simulink model "grid_afe_n"  (R2026a)
settings: Solver=ode23tb  StopTime=simlength  FixedStep=tc  MaxStep=glb_time.tc
values from neighbouring files (symbols this model uses):
  afe_ctrl = ctrl_afe_setup(glb_time.ts_afe, grid_emu.omega_grid_nom)    [init_model.m]
  afe_pwm_phase_shift_mod1 = 0    [init_model.m]
  afe_pwm_phase_shift_mod2 = 0    [init_model.m]
  afe_pwm_phase_shift_mod3 = 0    [init_model.m]
  afe_pwm_phase_shift_mod4 = 0    [init_model.m]
  filters = setup_global_filters(glb_time.ts_afe, glb_time.ts_inv, glb_time.ts_dab, glb_time.tc)    [init_model.m]
  frt_data = frt_settings(test_index, test_subindex, asymmetric_error_type,      enable_frt_1, enable_frt_2, start_time_LVRT, deepPOSxi, deepPOSeta, deepNEGxi, deepNEGeta)    [init_model.m]
  glb_time = timing_setup(fpwm_afe, trgo_afe, fpwm_inv, trgo_inv, fpwm_single_phase_inv, trgo_single_phase_inv, fpwm_dab, trgo_dab,      fpwm_psfbc, trgo_psfbc, fpwm_isop_rail, trgo_isop_rail, fpwm_cllc, trgo_cllc, t_measure, tc_factor, tc_decimation, delay_pwm, dead_time_afe,      dead_time_inv, dead_time_single_phase_inv, dead_time_dab, dead_time_psfbc, dead_time_isop_rail, dead_time_cllc)    [init_model.m]
  grid_emu = grid_three_phase_emulator('Dyn11', delta_star, grid_nominal_power, application_voltage, us1, us2, fgrid,                  eq_grid_inductance, eq_grid_resistance, eta, ucc, i1m, p_iron, n1, n2, core_area, core_length, mur,                  up_xi_pu_ref, up_eta_pu_ref, un_xi_pu_ref, un_eta_pu_ref)    [init_model.m]
  i_react_pos_ref_2 = -ixi_ref_mod1*tan(acos(0.95))    [init_model.m]
  i_react_pos_ref_3 = ixi_ref_mod1*tan(acos(0.95))    [init_model.m]
  ixi_ref_mod1 = -0.85    [init_model.m]
  ixi_ref_mod2 = -0.85    [init_model.m]
  ixi_ref_mod3 = -0.85    [init_model.m]
  ixi_ref_mod4 = -0.85    [init_model.m]
  ki_align = 18    [init_model.m]
  kp_align = 0.25    [init_model.m]
  lim_down_align = -0.05    [init_model.m]
  lim_up_align = 0.05    [init_model.m]
  mavarage_filter_frequency_base_order = 2    [init_model.m]
  time_gain_afe_module_1 = 1.0002    [init_model.m]
  time_gain_afe_module_2 = 1.0015    [init_model.m]
  time_gain_afe_module_3 = 0.9988    [init_model.m]
  time_gain_afe_module_4 = 1.0020    (= 1.002)    [init_model.m]
  time_i_react_pos_ref_1 = start_time_LVRT + error_length + 0.335    [init_model.m]
  time_i_react_pos_ref_2 = time_i_react_pos_ref_1 + 0.5    (= 0.5)    [init_model.m]
  u_cm_comp_mod1 = 0    [init_model.m]
  u_cm_comp_mod2 = -1    [init_model.m]
  u_cm_comp_mod3 = -1    [init_model.m]
  u_cm_comp_mod4 = -1    [init_model.m]
undefined symbols (not defined in the file or in its folder): hwdata, magnitude
libraries: fl_lib x113, nesl_utility x75, moving_average_filter x40, moving_average_filter_cc x32, sl_discontinuities x12, linear_double_integrator_observer_ccaller x8, discrete_time_low_pass_filter x4, threephase_inductor_lib x4, dclink_for_two_levels x4, three_phase_pwm_modulator x4, three_phase_inverter_ideal_switch_based_model x4, three_phase_inverter_igbt_advanced_thermal_model x4
(part 6 of 19)

== system grid_afe_n/afe_abc_mod3/AFE_control/afe_control/ig afe quantizzation and one step delay ==
  ig_abc_pu : Inport
  Demux1 : Demux  Outputs=3
  Mux1 : Mux  Inputs=3
  ig afe quantizzation and one step delay : Subsystem
  igd_abc_pu : Outport
  wires:
  Demux1/1 -> ig afe quantizzation and one step delay/1(ig_u_pu)
  Demux1/2 -> ig afe quantizzation and one step delay/2(ig_v_pu)
  ig_abc_pu/1 -> Demux1/1
  Mux1/1 -> igd_abc_pu/1
  Demux1/3 -> ig afe quantizzation and one step delay/3(ig_w_pu)
  ig afe quantizzation and one step delay/2(igd_v_pu) -> Mux1/2
  ig afe quantizzation and one step delay/1(igd_u_pu) -> Mux1/1
  ig afe quantizzation and one step delay/3(igd_w_pu) -> Mux1/3

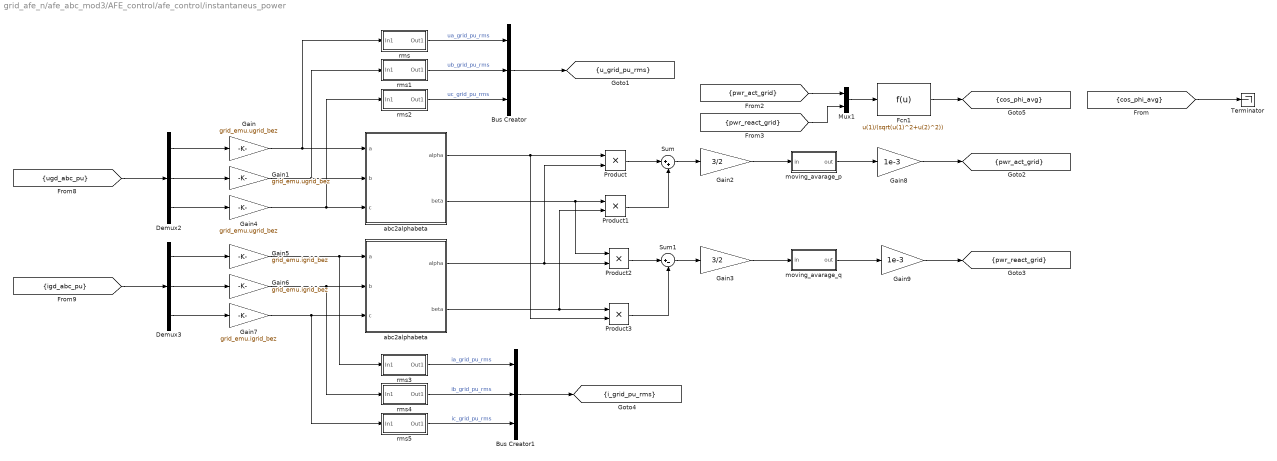
== system grid_afe_n/afe_abc_mod3/AFE_control/afe_control/instantaneus_power ==
  Bus Creator : BusCreator  Inputs=3
  Bus Creator1 : BusCreator  Inputs=3
  Demux2 : Demux  Outputs=3
  Demux3 : Demux  Outputs=3
  Fcn1 : Fcn  Expr=u(1)/(sqrt(u(1)^2+u(2)^2))
  Gain : Gain  Gain=grid_emu.ugrid_bez
  Gain1 : Gain  Gain=grid_emu.ugrid_bez
  Gain2 : Gain  Gain=3/2
  Gain3 : Gain  Gain=3/2
  Gain4 : Gain  Gain=grid_emu.ugrid_bez
  Gain5 : Gain  Gain=grid_emu.igrid_bez
  Gain6 : Gain  Gain=grid_emu.igrid_bez
  Gain7 : Gain  Gain=grid_emu.igrid_bez
  Gain8 : Gain  Gain=1e-3
  Gain9 : Gain  Gain=1e-3
  Mux1 : Mux  Inputs=2
  Product{,1..3} (4 alike) : Product  RndMeth=Zero
  Sum : Sum  Inputs=|++
  Sum1 : Sum  Inputs=|+-
  Terminator : Terminator
  abc2alphabeta : Subsystem
  "abc2alphabeta " : Subsystem
  moving_avarage_p : Subsystem
  moving_avarage_q : Subsystem
  rms : Subsystem
  rms1 : Subsystem
  rms2 : Subsystem
  rms3 : Subsystem
  rms4 : Subsystem
  rms5 : Subsystem
  tag scope: cos_phi_avg=scoped, i_grid_pu_rms=scoped, pwr_act_grid=scoped, pwr_react_grid=scoped, u_grid_pu_rms=scoped
  wires:
  abc2alphabeta/2("beta ") -> Product1/1, Product2/1
  "abc2alphabeta "/2("beta ") -> Product1/2, Product3/1
  abc2alphabeta/1("alpha ") -> Product3/2, Product/1
  "abc2alphabeta "/1("alpha ") -> Product2/2, Product/2
  Product/1 -> Sum/1
  Product1/1 -> Sum/2
  Product2/1 -> Sum1/1
  Product3/1 -> Sum1/2
  Sum1/1 -> Gain3/1
  Sum/1 -> Gain2/1
  Gain2/1 -> moving_avarage_p/1(in)
  Gain3/1 -> moving_avarage_q/1(in)
  [pwr_react_grid] -> Mux1/2
  Mux1/1 -> Fcn1/1
  Fcn1/1 -> [cos_phi_avg]
  [pwr_act_grid] -> Mux1/1
  rms/1(Out1) -> Bus Creator/1  "ua_grid_pu_rms"
  rms2/1(Out1) -> Bus Creator/3  "uc_grid_pu_rms"
  rms1/1(Out1) -> Bus Creator/2  "ub_grid_pu_rms"
  moving_avarage_p/1(out) -> Gain8/1
  moving_avarage_q/1(out) -> Gain9/1
  Demux2/1 -> Gain/1
  Demux2/2 -> Gain1/1
  Demux2/3 -> Gain4/1
  Demux3/1 -> Gain5/1
  Demux3/2 -> Gain6/1
  Demux3/3 -> Gain7/1
  Gain/1 -> rms/1(In1), abc2alphabeta/1(a)
  Gain1/1 -> rms1/1(In1), abc2alphabeta/2(b)
  Gain4/1 -> rms2/1(In1), abc2alphabeta/3(c)
  Gain5/1 -> rms3/1(In1), "abc2alphabeta "/1(a)
  Gain6/1 -> rms4/1(In1), "abc2alphabeta "/2(b)
  Gain7/1 -> rms5/1(In1), "abc2alphabeta "/3(c)
  Gain8/1 -> [pwr_act_grid]
  Gain9/1 -> [pwr_react_grid]
  [ugd_abc_pu] -> Demux2/1
  [igd_abc_pu] -> Demux3/1
  Bus Creator/1 -> [u_grid_pu_rms]
  rms4/1(Out1) -> Bus Creator1/2  "ib_grid_pu_rms"
  rms3/1(Out1) -> Bus Creator1/1  "ia_grid_pu_rms"
  rms5/1(Out1) -> Bus Creator1/3  "ic_grid_pu_rms"
  Bus Creator1/1 -> [i_grid_pu_rms]
  [cos_phi_avg] -> Terminator/1

== system grid_afe_n/afe_abc_mod3/AFE_control/afe_control/interesting scopes ==
  current_sequences_mod1 : Scope  NumInputPorts=4
      settings: ActiveDisplayYMinimum=-1.4062410671621262  ActiveDisplayYMaximum=0.648263540608363  DataLoggingVariableName=ScopeData2
  i_grid_seq_ref : Scope
      settings: ActiveDisplayYMinimum=-1.125  ActiveDisplayYMaximum=0.125
  voltage_sequences_mod1 : Scope  NumInputPorts=4
      settings: ActiveDisplayYMinimum=-1.2405151816982258  ActiveDisplayYMaximum=1.2605257614333911
  wires:
  [v_grid_neg_eta_avg] -> voltage_sequences_mod1/4  "u_grid_neg_eta"
  [i_grid_neg_xi_avg] -> current_sequences_mod1/3  "i_grid_neg_xi"
  [v_grid_pos_eta_avg] -> voltage_sequences_mod1/2  "u_grid_pos_eta"
  [v_grid_neg_xi_avg] -> voltage_sequences_mod1/3  "u_grid_neg_xi"
  [i_grid_pos_xi_avg] -> current_sequences_mod1/1  "i_grid_pos_xi"
  [i_grid_neg_eta_avg] -> current_sequences_mod1/4  "i_grid_neg_eta"
  [v_grid_pos_xi_avg] -> voltage_sequences_mod1/1  "u_grid_pos_xi"
  [i_grid_pos_eta_avg] -> current_sequences_mod1/2  "i_grid_pos_eta"
  [i_grid_seq_ref] -> i_grid_seq_ref/1  "i_grid_seq_ref"

== system grid_afe_n/afe_abc_mod3/AFE_control/afe_control/is afe quantizzation and one step delay ==
  is_abc_pu : Inport
  Demux : Demux  Outputs=3
  Mux : Mux  Inputs=3
  is afe quantizzation and one step delay : Subsystem
  isd_abc_pu : Outport
  wires:
  is afe quantizzation and one step delay/2(isd_v_pu) -> Mux/2
  is_abc_pu/1 -> Demux/1
  is afe quantizzation and one step delay/3(isd_w_pu) -> Mux/3
  is afe quantizzation and one step delay/1(isd_u_pu) -> Mux/1
  Demux/1 -> is afe quantizzation and one step delay/1(is_u_pu)
  Mux/1 -> isd_abc_pu/1
  Demux/3 -> is afe quantizzation and one step delay/3(is_w_pu)
  Demux/2 -> is afe quantizzation and one step delay/2(is_v_pu)

== system grid_afe_n/afe_abc_mod3/AFE_control/afe_control/islanding_mode_detector ==
  gamma : Inport
  alpha : Inport  Port=2
  beta : Inport  Port=3
  Gain : Gain  Gain=7
  MATLAB Function : MATLAB Function  TreatAsAtomicUnit=on
  Terminator : Terminator
  Terminator1 : Terminator
  bounder : MATLAB Function  TreatAsAtomicUnit=on
  moving_avarage_1 : Subsystem
  moving_avarage_2 : Subsystem
  seventh_ugrid_component : Scope  NumInputPorts=2
      settings: ActiveDisplayYMinimum=-0.0034745064787606167  ActiveDisplayYMaximum=0.0074022094547510631  DataLoggingVariableName=ScopeData10
  tag scope: u_7th_eta_avg=scoped, u_7th_xi_avg=scoped
  wires:
  gamma/1 -> Gain/1  "gamma_grid"
  MATLAB Function/1(xi) -> moving_avarage_1/1(u)
  bounder/1(y) -> MATLAB Function/3(gamma)
  Gain/1 -> bounder/1(u)
  alpha/1 -> MATLAB Function/1(alpha)  "u_grid_alpha"
  beta/1 -> MATLAB Function/2(beta)  "u_grid_beta"
  MATLAB Function/2(eta) -> moving_avarage_2/1(u)
  moving_avarage_1/1(y) -> [u_7th_xi_avg], seventh_ugrid_component/1  "u_7th_xi"
  moving_avarage_2/1(y) -> seventh_ugrid_component/2, [u_7th_eta_avg]  "u_7th_eta"
  [u_7th_xi_avg] -> Terminator/1
  [u_7th_eta_avg] -> Terminator1/1

== system grid_afe_n/afe_abc_mod3/AFE_control/afe_control/phase_compensation_1 ==
  local_time : Inport
  master_time : Inport  Port=2
  Zero-Order Hold : ZeroOrderHold  SampleTime=-1
  Zero-Order Hold1 : ZeroOrderHold  SampleTime=-1
  alignment_eval_afe1 : Subsystem
  y : Outport
  wires:
  local_time/1 -> Zero-Order Hold/1
  master_time/1 -> Zero-Order Hold1/1
  alignment_eval_afe1/1(dp) -> y/1
  Zero-Order Hold/1 -> alignment_eval_afe1/1(local_time)
  Zero-Order Hold1/1 -> alignment_eval_afe1/2(master_time)

== system grid_afe_n/afe_abc_mod3/AFE_control/afe_control/space_vector ==
  uab_out : Inport
  Bus Creator : BusCreator  Inputs=3
  Bus Selector : BusSelector  OutputSignals=da,db,dc
  Bus Selector1 : BusSelector  OutputSignals=ualpha_afe,ubeta_afe,ugamma_afe
  C Caller : CCaller  FunctionName=sv_pwm_cm_process_simulink  PortSpecificationStruct="%)30     .    B H   8    (     @         %    \"     8    !     0         %  0 \"0    $    _    07)G3F%M90  4&]R=$YA;64 4V-O<&4     26YD97@     5'EP90      4VEZ90      27-';&]B86P   X    P    !@    @    $          4    (     0    ,    !         !   P!O=70 #@   #     &    \"     0         !0    @    !     P    $         $  # &]U=  .    .     8    (    !          %    \"     $    &     0         0   ...(+3252 chars)"
  Constant : Constant  Value=glb_time.ts_afe
  Constant1 : Constant
  Data Type Conversion1 : DataTypeConversion  OutDataTypeStr=double  SaturateOnIntegerOverflow=off  RndMeth=Floor
  Data Type Conversion{4,15..16,18} (4 alike) : DataTypeConversion  OutDataTypeStr=single  SaturateOnIntegerOverflow=off  RndMeth=Floor
  Data Type Conversion17 : DataTypeConversion  OutDataTypeStr=uint32  SaturateOnIntegerOverflow=off  RndMeth=Floor
  Data Type Conversion2 : DataTypeConversion  OutDataTypeStr=double  SaturateOnIntegerOverflow=off  RndMeth=Floor
  Data Type Conversion3 : DataTypeConversion  OutDataTypeStr=double  SaturateOnIntegerOverflow=off  RndMeth=Floor
  Gain1 : Gain  Gain=sqrt(3)/2
  Gain2 : Gain  Gain=sqrt(3)/2
  Gain3 : Gain  Gain=u_cm_comp_mod3
  duvw : Outport
  wires:
  Data Type Conversion15/1 -> C Caller/2
  Bus Selector/2 -> Data Type Conversion2/1  "<db>"
  Data Type Conversion18/1 -> C Caller/1
  C Caller/1 -> Bus Selector/1
  Bus Creator/1 -> duvw/1
  Data Type Conversion1/1 -> Bus Creator/1  "du(k)"
  Bus Selector1/2 -> Gain2/1  "<ubeta_afe>"
  Bus Selector/3 -> Data Type Conversion3/1  "<dc>"
  Bus Selector1/1 -> Gain1/1  "<ualpha_afe>"
  Data Type Conversion2/1 -> Bus Creator/2  "dv(k)"
  Gain2/1 -> Data Type Conversion15/1
  Bus Selector/1 -> Data Type Conversion1/1  "<da>"
  Gain1/1 -> Data Type Conversion18/1
  Data Type Conversion3/1 -> Bus Creator/3  "dw(k)"
  Constant/1 -> Data Type Conversion16/1
  uab_out/1 -> Bus Selector1/1
  Constant1/1 -> Data Type Conversion17/1
  Data Type Conversion16/1 -> C Caller/4
  Data Type Conversion17/1 -> C Caller/5
  Bus Selector1/3 -> Gain3/1  "<ugamma_afe>"
  Gain3/1 -> Data Type Conversion4/1
  Data Type Conversion4/1 -> C Caller/3

== system grid_afe_n/afe_abc_mod3/AFE_control/afe_control/udc_acquisition ==
  udc_pu : Inport
  Quantizer : Quantizer  QuantizationInterval=adc_quantization
  Unit Delay : UnitDelay  SampleTime=-1
  Zero-Order Hold : ZeroOrderHold  SampleTime=-1
  udcd_pu : Outport
  wires:
  Quantizer/1 -> Unit Delay/1
  udc_pu/1 -> Zero-Order Hold/1
  Unit Delay/1 -> udcd_pu/1
  Zero-Order Hold/1 -> Quantizer/1

== system grid_afe_n/afe_abc_mod3/AFE_control/afe_control/udc_ctrl ==
  udc_pu : Inport
  udc_pu_ref : Inport  Port=2
  1/Ti : Gain  Gain=afe_ctrl.kp_udc_ctrl  SaturateOnIntegerOverflow=on  OutDataTypeStr=Inherit: Same as input  ParamDataTypeStr=Inherit: Same as input
  Constant : Constant  Value=0
  Gain : Gain  Gain=-1
  Saturation : Saturate  UpperLimit=afe_ctrl.ixi_pos_ref_lim  LowerLimit=-afe_ctrl.ixi_pos_ref_lim
  Sum1 : Sum  Inputs=+++  SaturateOnIntegerOverflow=on
  Sum2 : Sum  Inputs=-+  SaturateOnIntegerOverflow=on
  Sum3 : Sum  Inputs=-+  SaturateOnIntegerOverflow=on
  Switch : Switch  Criteria=u2 > Threshold  SaturateOnIntegerOverflow=off  InputSameDT=off
  To Workspace1 : ToWorkspace  VariableName=udc_pu_sim_mod1  SampleTime=-1
      settings: MaxDataPoints=glb_time.Ns_afe
  To Workspace3 : ToWorkspace  VariableName=udc_pu_ref_sim_mod1  SampleTime=-1
      settings: MaxDataPoints=glb_time.Ns_afe
  Unit Delay4 : UnitDelay  SampleTime=-1
  kp : Gain  Gain=afe_ctrl.ki_udc_ctrl*glb_time.ts_afe  SaturateOnIntegerOverflow=on  OutDataTypeStr=Inherit: Same as input  ParamDataTypeStr=Inherit: Same as input
  udc_tracking : Scope  NumInputPorts=2
      settings: ActiveDisplayYMinimum=-0.14752197265624997  ActiveDisplayYMaximum=1.32769775390625  DataLoggingVariableName=ScopeData8
  i_xi_ref : Outport
  wires:
  1/Ti/1 -> Sum1/1, Sum3/1
  kp/1 -> Sum1/2
  Sum3/1 -> Unit Delay4/1
  Unit Delay4/1 -> Sum1/3
  udc_pu_ref/1 -> To Workspace3/1, udc_tracking/1, Sum2/2  "udc_pu_ref"
  udc_pu/1 -> To Workspace1/1, udc_tracking/2, Sum2/1  "udc_pu"
  Sum2/1 -> kp/1, 1/Ti/1
  Sum1/1 -> Saturation/1
  [pwr_lim_enable] -> Switch/2
  Saturation/1 -> Switch/3
  Switch/1 -> Sum3/2, Gain/1
  Constant/1 -> Switch/1
  Gain/1 -> i_xi_ref/1

== system grid_afe_n/afe_abc_mod3/AFE_control/afe_control/ug afe quantizzation and one step delay ==
  ug_abc_pu : Inport
  Demux : Demux  Outputs=3
  Mux : Mux  Inputs=3
  ug afe quantizzation and one step delay : Subsystem
  ugd_abc_pu : Outport
  wires:
  ug afe quantizzation and one step delay/2(ugd_v_pu) -> Mux/2
  Demux/2 -> ug afe quantizzation and one step delay/2(ug_v_pu)
  Demux/3 -> ug afe quantizzation and one step delay/3(ug_w_pu)
  ug afe quantizzation and one step delay/1(ugd_u_pu) -> Mux/1
  Demux/1 -> ug afe quantizzation and one step delay/1(ug_u_pu)
  ug_abc_pu/1 -> Demux/1
  ug afe quantizzation and one step delay/3(ugd_w_pu) -> Mux/3
  Mux/1 -> ugd_abc_pu/1

== system grid_afe_n/afe_abc_mod3/afe/sv_pwm/modulator1 ==
  u : Inport
  v : Inport  Port=2
  w : Inport  Port=3
  phase : Inport  Port=4
  Bus Creator : BusCreator  Inputs=3
  Three phase two level PWM generator with global TRGO : three_phase_pwm_modulator/Three phase two level PWM generator with global TRGO  f=glb_time.fPWM_AFE  m_up=0.98  m_low=0.02  dead_time=glb_time.dead_time_AFE  pos_cmd_gate=15  neg_cmd_gate=-10  polarity=1  tc=glb_time.tc  double_sampling=1
      link override gate commands/Bus Selector: OutputSignals=du(t)
      link override gate commands/Bus Selector1: OutputSignals=dv(t)
      link override gate commands/Bus Selector2: OutputSignals=dw(t)
  gate_cmds : Outport
  tag scope: TRGO_afe_module_3=global
  wires:
  [time_afe_module_3] -> Three phase two level PWM generator with global TRGO/1
  Bus Creator/1 -> Three phase two level PWM generator with global TRGO/3
  Three phase two level PWM generator with global TRGO/1 -> [TRGO_afe_module_3]
  u/1 -> Bus Creator/1
  v/1 -> Bus Creator/2
  w/1 -> Bus Creator/3
  phase/1 -> Three phase two level PWM generator with global TRGO/2
  Three phase two level PWM generator with global TRGO/2 -> gate_cmds/1

== system grid_afe_n/afe_abc_mod4/AFE_control/afe_control/FRT-VDE4110 ==
  Constant : Constant  Value=0
  FRT-Detection : Subsystem
  FRT-PosNegReactiveCurrentReferences : Subsystem
  Terminator : Terminator
  Terminator1 : Terminator
  frt_detection_output : Scope  NumInputPorts=3
      settings: ActiveDisplayYMinimum=-1  ActiveDisplayYMaximum=1
  tag scope: frt_active=scoped, pwr_lim_enable=scoped
  wires:
  FRT-Detection/2(frt_state) -> frt_detection_output/1  "frt_state"
  FRT-Detection/5(pwr_lim_enable) -> [pwr_lim_enable], frt_detection_output/3  "pwr_lim_enable"
  FRT-Detection/4(frt_active) -> [frt_active], frt_detection_output/2  "frt_active"
  [v_grid_pos_eta_avg] -> FRT-PosNegReactiveCurrentReferences/2(In2)
  [v_grid_neg_eta_avg] -> FRT-PosNegReactiveCurrentReferences/4(In4)
  [v_grid_neg_xi_avg] -> FRT-PosNegReactiveCurrentReferences/3(In3)
  [v_grid_pos_xi_avg] -> FRT-PosNegReactiveCurrentReferences/1(In1)
  Constant/1 -> FRT-Detection/1(red_dyn_enabled)
  FRT-Detection/1(frt_exceeded) -> Terminator/1
  FRT-Detection/3(red_dyn_active) -> Terminator1/1

== system grid_afe_n/afe_abc_mod4/AFE_control/afe_control/current_ctrl ==
  i_xi_ref : Inport
  Demux : Demux  Outputs=3
  current_transformation : Subsystem
  inner_current_ctrl : Subsystem
  xieta2abc : Subsystem
  uabg_out : Outport
  wires:
  [i_stack_pos_eta_ref] -> xieta2abc/2(pos_eta)
  [i_stack_neg_xi_ref] -> xieta2abc/3(neg_xi)
  [i_stack_neg_eta_ref] -> xieta2abc/4(neg_eta)
  i_xi_ref/1 -> xieta2abc/1(pos_xi)  "i_xi_ref"
  inner_current_ctrl/1(uabg) -> uabg_out/1
  [isd_abc_pu] -> inner_current_ctrl/2(is_abc)
  xieta2abc/1(i_abc) -> inner_current_ctrl/1(In1)
  [phase_grid_pll] -> xieta2abc/5(phase)
  [isd_abc_pu] -> Demux/1
  Demux/3 -> current_transformation/3(is_c_pu)  "is_c"
  Demux/2 -> current_transformation/2(is_b_pu)  "is_b"
  Demux/1 -> current_transformation/1(is_a_pu)  "is_a"

== system grid_afe_n/afe_abc_mod4/AFE_control/afe_control/data_to_worspace_module_1 ==
  Bus Creator : BusCreator  Inputs=5
  dq_pll : Subsystem
  inner_current_tracking : Subsystem
  pwr_meter : Subsystem
  sequences_data : Subsystem
  m : Outport
  wires:
  [local_time] -> Bus Creator/5  "local_time"
  inner_current_tracking/1(m_inner_current_tracking) -> Bus Creator/3  "inner_current_tracking"
  pwr_meter/1(m_pwr_meter) -> Bus Creator/2  "pwr_meter"
  sequences_data/1(m_seq) -> Bus Creator/1  "sequences_data"
  Bus Creator/1 -> m/1
  dq_pll/1(dqPLLs) -> Bus Creator/4  "dq_pll"

== system grid_afe_n/afe_abc_mod4/AFE_control/afe_control/grid_current_sequences_and_reactive_pwr_ctrl ==
  ig_abc_pu : Inport
  current_sequence_avg : Subsystem
  grid_current_sampling_and_alpha_beta_transformation : Subsystem
  i_alphabeta2xieta : Subsystem
  sequences_current_control : Subsystem
  tag scope: i_grid_neg_eta_avg=scoped, i_grid_neg_xi_avg=scoped, i_grid_pos_eta_avg=scoped, i_grid_pos_xi_avg=scoped
  wires:
  current_sequence_avg/3(i_grid_neg_xi_avg) -> [i_grid_neg_xi_avg], sequences_current_control/3(i_neg_xi)
  grid_current_sampling_and_alpha_beta_transformation/1(i_grid_alpha) -> i_alphabeta2xieta/1(alpha)
  grid_current_sampling_and_alpha_beta_transformation/2(i_grid_beta) -> i_alphabeta2xieta/2(beta)
  [phase_grid_pll] -> i_alphabeta2xieta/3(gamma)
  current_sequence_avg/2(i_grid_pos_eta_avg) -> sequences_current_control/2(i_pos_eta), [i_grid_pos_eta_avg]
  current_sequence_avg/1(i_grid_pos_xi_avg) -> sequences_current_control/1(i_pos_xi), [i_grid_pos_xi_avg]
  i_alphabeta2xieta/2(v_grid_pos_eta) -> current_sequence_avg/2(i_grid_pos_eta)
  ig_abc_pu/1 -> grid_current_sampling_and_alpha_beta_transformation/1(ig_abc)
  current_sequence_avg/4(i_grid_neg_eta_avg) -> [i_grid_neg_eta_avg], sequences_current_control/4(i_neg_eta)
  i_alphabeta2xieta/4(e) -> current_sequence_avg/4(i_grid_neg_eta)
  i_alphabeta2xieta/3(v_grid_neg_xi) -> current_sequence_avg/3(i_grid_neg_xi)
  i_alphabeta2xieta/1(xi) -> current_sequence_avg/1(i_grid_pos_xi)

== system grid_afe_n/afe_abc_mod4/AFE_control/afe_control/grid_phase_acquisition ==
  grid_phase : Inport
  Quantizer : Quantizer  QuantizationInterval=adc_quantization
  Unit Delay : UnitDelay  SampleTime=-1
  Zero-Order Hold : ZeroOrderHold  SampleTime=-1
  grid_phased : Outport
  wires:
  Quantizer/1 -> Unit Delay/1
  grid_phase/1 -> Zero-Order Hold/1
  Unit Delay/1 -> grid_phased/1
  Zero-Order Hold/1 -> Quantizer/1

== system grid_afe_n/afe_abc_mod4/AFE_control/afe_control/grid_voltage_phase_lock_loops ==
  ug_abc_pu : Inport
  Bus Creator : BusCreator  Inputs=5
  Bus Creator1 : BusCreator  Inputs=4
  Bus Creator2 : BusCreator  Inputs=2
  FHT-PLL : Subsystem  Commented=on
  FHT-PLL performance : Scope  NumInputPorts=2
      settings: ActiveDisplayYMinimum=-1.251220703125  ActiveDisplayYMaximum=1.251220703125  DataLoggingVariableName=ScopeData8
  FHT-PLL_simulink : Subsystem
  Variant Source1 : VariantSource  VariantControls={use_dq_pll_mode1_modn == 1, use_dq_pll_mode2_modn == 1, use_dq_pll_mode3_modn == 1, use_dq_pll_mode4_modn == 1}
  Variant Source2 : VariantSource  VariantControls={use_dq_pll_mode1_modn == 1, use_dq_pll_mode2_modn == 1, use_dq_pll_mode3_modn == 1, use_dq_pll_mode4_modn == 1}
  dq_pll : Subsystem
  dq_pll_ccaller : Subsystem  Commented=on
  dqpll_ccaler : Scope  Commented=on  NumInputPorts=3
      settings: ActiveDisplayYMinimum=-0.88802937790751446  ActiveDisplayYMaximum=4.5431143753230572  DataLoggingVariableName=ScopeData4
  pll_performances : Scope  NumInputPorts=2
      settings: ActiveDisplayYMinimum=-3.7285036241199436  ActiveDisplayYMaximum=4.0550847544280391  DataLoggingVariableName=ScopeData34
  tag scope: omega_grid_dqpll_ccaller=scoped, omega_grid_fht_simulink_pll=scoped, omega_grid_fhtsr_dqpll=scoped, omega_grid_pll_pu=scoped, omega_grid_pu_dqpll=scoped, phase_grid_dqpll=scoped, phase_grid_dqpll_ccaller=scoped, phase_grid_fht_simulink_pll=scoped, phase_grid_fhtsr_dqpll=scoped, phase_grid_pll=scoped
  wires:
  [phase_grid_fhtsr_dqpll] -> Bus Creator2/1  "phase_grid_fht_pll"
  [omega_grid_fhtsr_dqpll] -> Bus Creator2/2  "omega_grid_fht_pll"
  Bus Creator2/1 -> FHT-PLL performance/2
  [omega_grid_fhtsr_dqpll] -> Variant Source2/4  "omega_grid_fht_pll"
  [phase_grid_fhtsr_dqpll] -> Variant Source1/4  "phase_grid_fht_pll"
  [omega_grid_fhtsr_dqpll] -> Bus Creator1/4  "omega_grid_fht_pll"
  [phase_grid_fhtsr_dqpll] -> Bus Creator/5  "phase_grid_fht_pll"
  FHT-PLL/1(gamma_grid_fht_pll) -> [phase_grid_fhtsr_dqpll]
  FHT-PLL/2(omega_grid_fht_pll) -> [omega_grid_fhtsr_dqpll]
  [grid_emulator_phase] -> Bus Creator/4  "grid_emulator_phase"
  Bus Creator1/1 -> pll_performances/2
  Bus Creator/1 -> pll_performances/1
  ug_abc_pu/1 -> dq_pll_ccaller/1(ug_abc_pu), FHT-PLL_simulink/1(ug_abc_pu), FHT-PLL/1(ug_abc_pu), dq_pll/1(ug_abc_pu), FHT-PLL performance/1
  dq_pll_ccaller/5(dqpll_state) -> dqpll_ccaler/3  "dqpll_state"
  dq_pll_ccaller/4(dqpll_ueta) -> dqpll_ccaler/2  "ueta_n"
  dq_pll_ccaller/3(dqpll_uxi) -> dqpll_ccaler/1  "uxi_n"
  Variant Source2/1 -> [omega_grid_pll_pu]
  [omega_grid_fht_simulink_pll] -> Variant Source2/3, Bus Creator1/3  "omega_grid_fht_simulink_pll"
  [omega_grid_dqpll_ccaller] -> Variant Source2/2, Bus Creator1/2  "omega_grid_dqpll_ccaller"
  [omega_grid_pu_dqpll] -> Variant Source2/1, Bus Creator1/1  "omega_grid_pu_dqpll"
  [phase_grid_fht_simulink_pll] -> Variant Source1/3, Bus Creator/3  "phase_grid_fht_simulink_pll"
  [phase_grid_dqpll_ccaller] -> Variant Source1/2, Bus Creator/2  "phase_grid_dqpll_ccaller"
  [phase_grid_dqpll] -> Bus Creator/1, Variant Source1/1  "phase_grid_dqpll"
  dq_pll_ccaller/2(omega_pu_hat) -> [omega_grid_dqpll_ccaller]
  dq_pll_ccaller/1(gamma_hat) -> [phase_grid_dqpll_ccaller]
  dq_pll/1(phase_grid_dqpll) -> [phase_grid_dqpll]
  dq_pll/2(omega_grid_pu_dqpll) -> [omega_grid_pu_dqpll]
  Variant Source1/1 -> [phase_grid_pll]
  FHT-PLL_simulink/1(gamma_grid_fht_pll) -> [phase_grid_fht_simulink_pll]
  FHT-PLL_simulink/2(omega_grid_fht_pll) -> [omega_grid_fht_simulink_pll]

== system grid_afe_n/afe_abc_mod4/AFE_control/afe_control/grid_voltage_sequences ==
  grid_voltage_sampling_and_alpha_beta_transformation : Subsystem
  v_alphabeta2xieta : Subsystem
  voltage_sequence_avg : Subsystem
  tag scope: ug_alpha_pu=scoped, ug_beta_pu=scoped, v_grid_neg_eta_avg=scoped, v_grid_neg_xi_avg=scoped, v_grid_pos_eta_avg=scoped, v_grid_pos_xi_avg=scoped
  wires:
  [ugd_abc_pu] -> grid_voltage_sampling_and_alpha_beta_transformation/1(v_abc)
  grid_voltage_sampling_and_alpha_beta_transformation/1(u_grid_alpha) -> v_alphabeta2xieta/1(alpha), [ug_alpha_pu]
  v_alphabeta2xieta/1(xi) -> voltage_sequence_avg/1(v_grid_pos_xi)  "pos_xi"
  voltage_sequence_avg/1(v_grid_pos_xi_avg) -> [v_grid_pos_xi_avg]
  grid_voltage_sampling_and_alpha_beta_transformation/2(u_grid_beta) -> v_alphabeta2xieta/2(beta), [ug_beta_pu]
  voltage_sequence_avg/4(v_grid_neg_eta_avg) -> [v_grid_neg_eta_avg]
  voltage_sequence_avg/2(v_grid_pos_eta_avg) -> [v_grid_pos_eta_avg]
  voltage_sequence_avg/3(v_grid_neg_xi_avg) -> [v_grid_neg_xi_avg]
  v_alphabeta2xieta/3(v_grid_neg_xi) -> voltage_sequence_avg/3(v_grid_neg_xi)  "neg_xi"
  [phase_grid_pll] -> v_alphabeta2xieta/3(gamma)
  v_alphabeta2xieta/2(eta) -> voltage_sequence_avg/2(v_grid_pos_eta)  "pos_eta"
  v_alphabeta2xieta/4(v_grid_neg_eta) -> voltage_sequence_avg/4(v_grid_neg_eta)  "neg_eta"

== system grid_afe_n/afe_abc_mod4/AFE_control/afe_control/i_xi_ref ==
  Constant1 : Constant  Value=ixi_ref_mod4
  Constant2 : Constant  Value=0
  Delay : Delay  DelayLength=floor(0.25/glb_time.ts_afe)
  Switch : Switch  Criteria=u2 > Threshold  SaturateOnIntegerOverflow=off  InputSameDT=off
  Switch1 : Switch  Criteria=u2 > Threshold  SaturateOnIntegerOverflow=off  InputSameDT=off
  Variant Source : VariantSource  VariantControls={false, true}
  discrete-time-low-pass-filter : discrete_time_low_pass_filter/discrete-time-low-pass-filter  tau=0.125  ts=glb_time.ts_afe
  i_xi_ref : Outport
  wires:
  Constant1/1 -> Switch/3  "i_xi_ref"
  Constant2/1 -> Switch/1
  [pwr_lim_enable] -> Switch/2
  [pwr_lim_enable] -> Delay/1
  Switch/1 -> discrete-time-low-pass-filter/1, Variant Source/2, Switch1/3
  Delay/1 -> Switch1/2
  discrete-time-low-pass-filter/1 -> Switch1/1
  Switch1/1 -> Variant Source/1
  Variant Source/1 -> i_xi_ref/1

== system grid_afe_n/afe_abc_mod4/AFE_control/afe_control/ig afe quantizzation and one step delay ==
  ig_abc_pu : Inport
  Demux1 : Demux  Outputs=3
  Mux1 : Mux  Inputs=3
  ig afe quantizzation and one step delay : Subsystem
  igd_abc_pu : Outport
  wires:
  ig afe quantizzation and one step delay/3(igd_w_pu) -> Mux1/3
  ig afe quantizzation and one step delay/1(igd_u_pu) -> Mux1/1
  ig afe quantizzation and one step delay/2(igd_v_pu) -> Mux1/2
  Demux1/3 -> ig afe quantizzation and one step delay/3(ig_w_pu)
  Mux1/1 -> igd_abc_pu/1
  ig_abc_pu/1 -> Demux1/1
  Demux1/2 -> ig afe quantizzation and one step delay/2(ig_v_pu)
  Demux1/1 -> ig afe quantizzation and one step delay/1(ig_u_pu)

== system grid_afe_n/afe_abc_mod4/AFE_control/afe_control/instantaneus_power ==
  Bus Creator : BusCreator  Inputs=3
  Bus Creator1 : BusCreator  Inputs=3
  Demux2 : Demux  Outputs=3
  Demux3 : Demux  Outputs=3
  Fcn1 : Fcn  Expr=u(1)/(sqrt(u(1)^2+u(2)^2))
  Gain : Gain  Gain=grid_emu.ugrid_bez
  Gain1 : Gain  Gain=grid_emu.ugrid_bez
  Gain2 : Gain  Gain=3/2
  Gain3 : Gain  Gain=3/2
  Gain4 : Gain  Gain=grid_emu.ugrid_bez
  Gain5 : Gain  Gain=grid_emu.igrid_bez
  Gain6 : Gain  Gain=grid_emu.igrid_bez
  Gain7 : Gain  Gain=grid_emu.igrid_bez
  Gain8 : Gain  Gain=1e-3
  Gain9 : Gain  Gain=1e-3
  Mux1 : Mux  Inputs=2
  Product{,1..3} (4 alike) : Product  RndMeth=Zero
  Sum : Sum  Inputs=|++
  Sum1 : Sum  Inputs=|+-
  Terminator : Terminator
  abc2alphabeta : Subsystem
  "abc2alphabeta " : Subsystem
  moving_avarage_p : Subsystem
  moving_avarage_q : Subsystem
  rms : Subsystem
  rms1 : Subsystem
  rms2 : Subsystem
  rms3 : Subsystem
  rms4 : Subsystem
  rms5 : Subsystem
  tag scope: cos_phi_avg=scoped, i_grid_pu_rms=scoped, pwr_act_grid=scoped, pwr_react_grid=scoped, u_grid_pu_rms=scoped
  wires:
  Bus Creator1/1 -> [i_grid_pu_rms]
  rms5/1(Out1) -> Bus Creator1/3  "ic_grid_pu_rms"
  rms3/1(Out1) -> Bus Creator1/1  "ia_grid_pu_rms"
  rms4/1(Out1) -> Bus Creator1/2  "ib_grid_pu_rms"
  Bus Creator/1 -> [u_grid_pu_rms]
  [igd_abc_pu] -> Demux3/1
  [ugd_abc_pu] -> Demux2/1
  Gain9/1 -> [pwr_react_grid]
  Gain8/1 -> [pwr_act_grid]
  Gain7/1 -> "abc2alphabeta "/3(c), rms5/1(In1)
  Gain6/1 -> "abc2alphabeta "/2(b), rms4/1(In1)
  Gain5/1 -> "abc2alphabeta "/1(a), rms3/1(In1)
  Gain4/1 -> abc2alphabeta/3(c), rms2/1(In1)
  Gain1/1 -> abc2alphabeta/2(b), rms1/1(In1)
  Gain/1 -> abc2alphabeta/1(a), rms/1(In1)
  Demux3/3 -> Gain7/1
  Demux3/2 -> Gain6/1
  Demux3/1 -> Gain5/1
  Demux2/3 -> Gain4/1
  Demux2/2 -> Gain1/1
  Demux2/1 -> Gain/1
  moving_avarage_q/1(out) -> Gain9/1
  moving_avarage_p/1(out) -> Gain8/1
  rms1/1(Out1) -> Bus Creator/2  "ub_grid_pu_rms"
  rms2/1(Out1) -> Bus Creator/3  "uc_grid_pu_rms"
  rms/1(Out1) -> Bus Creator/1  "ua_grid_pu_rms"
  [pwr_act_grid] -> Mux1/1
  Fcn1/1 -> [cos_phi_avg]
  Mux1/1 -> Fcn1/1
  [pwr_react_grid] -> Mux1/2
  Gain3/1 -> moving_avarage_q/1(in)
  Gain2/1 -> moving_avarage_p/1(in)
  Sum/1 -> Gain2/1
  Sum1/1 -> Gain3/1
  Product3/1 -> Sum1/2
  Product2/1 -> Sum1/1
  Product1/1 -> Sum/2
  Product/1 -> Sum/1
  "abc2alphabeta "/1("alpha ") -> Product/2, Product2/2
  abc2alphabeta/1("alpha ") -> Product/1, Product3/2
  "abc2alphabeta "/2("beta ") -> Product3/1, Product1/2
  abc2alphabeta/2("beta ") -> Product2/1, Product1/1
  [cos_phi_avg] -> Terminator/1

== system grid_afe_n/afe_abc_mod4/AFE_control/afe_control/interesting scopes ==
  current_sequences_mod1 : Scope  NumInputPorts=4
      settings: ActiveDisplayYMinimum=-1.4062410671621262  ActiveDisplayYMaximum=0.648263540608363  DataLoggingVariableName=ScopeData2
  i_grid_seq_ref : Scope
      settings: ActiveDisplayYMinimum=-1.125  ActiveDisplayYMaximum=0.125
  voltage_sequences_mod1 : Scope  NumInputPorts=4
      settings: ActiveDisplayYMinimum=-1.2405151816982258  ActiveDisplayYMaximum=1.2605257614333911
  wires:
  [i_grid_seq_ref] -> i_grid_seq_ref/1  "i_grid_seq_ref"
  [i_grid_pos_eta_avg] -> current_sequences_mod1/2  "i_grid_pos_eta"
  [v_grid_pos_xi_avg] -> voltage_sequences_mod1/1  "u_grid_pos_xi"
  [i_grid_neg_eta_avg] -> current_sequences_mod1/4  "i_grid_neg_eta"
  [i_grid_pos_xi_avg] -> current_sequences_mod1/1  "i_grid_pos_xi"
  [v_grid_neg_xi_avg] -> voltage_sequences_mod1/3  "u_grid_neg_xi"
  [v_grid_pos_eta_avg] -> voltage_sequences_mod1/2  "u_grid_pos_eta"
  [i_grid_neg_xi_avg] -> current_sequences_mod1/3  "i_grid_neg_xi"
  [v_grid_neg_eta_avg] -> voltage_sequences_mod1/4  "u_grid_neg_eta"

== system grid_afe_n/afe_abc_mod4/AFE_control/afe_control/is afe quantizzation and one step delay ==
  is_abc_pu : Inport
  Demux : Demux  Outputs=3
  Mux : Mux  Inputs=3
  is afe quantizzation and one step delay : Subsystem
  isd_abc_pu : Outport
  wires:
  Demux/2 -> is afe quantizzation and one step delay/2(is_v_pu)
  Demux/3 -> is afe quantizzation and one step delay/3(is_w_pu)
  Mux/1 -> isd_abc_pu/1
  Demux/1 -> is afe quantizzation and one step delay/1(is_u_pu)
  is afe quantizzation and one step delay/1(isd_u_pu) -> Mux/1
  is afe quantizzation and one step delay/3(isd_w_pu) -> Mux/3
  is_abc_pu/1 -> Demux/1
  is afe quantizzation and one step delay/2(isd_v_pu) -> Mux/2

== system grid_afe_n/afe_abc_mod4/AFE_control/afe_control/islanding_mode_detector ==
  gamma : Inport
  alpha : Inport  Port=2
  beta : Inport  Port=3
  Gain : Gain  Gain=7
  MATLAB Function : MATLAB Function  TreatAsAtomicUnit=on
  Terminator : Terminator
  Terminator1 : Terminator
  bounder : MATLAB Function  TreatAsAtomicUnit=on
  moving_avarage_1 : Subsystem
  moving_avarage_2 : Subsystem
  seventh_ugrid_component : Scope  NumInputPorts=2
      settings: ActiveDisplayYMinimum=-0.0034745064787606167  ActiveDisplayYMaximum=0.0074022094547510631  DataLoggingVariableName=ScopeData10
  tag scope: u_7th_eta_avg=scoped, u_7th_xi_avg=scoped
  wires:
  moving_avarage_2/1(y) -> seventh_ugrid_component/2, [u_7th_eta_avg]  "u_7th_eta"
  moving_avarage_1/1(y) -> seventh_ugrid_component/1, [u_7th_xi_avg]  "u_7th_xi"
  MATLAB Function/2(eta) -> moving_avarage_2/1(u)
  beta/1 -> MATLAB Function/2(beta)  "u_grid_beta"
  alpha/1 -> MATLAB Function/1(alpha)  "u_grid_alpha"
  Gain/1 -> bounder/1(u)
  bounder/1(y) -> MATLAB Function/3(gamma)
  MATLAB Function/1(xi) -> moving_avarage_1/1(u)
  gamma/1 -> Gain/1  "gamma_grid"
  [u_7th_xi_avg] -> Terminator/1
  [u_7th_eta_avg] -> Terminator1/1

== system grid_afe_n/afe_abc_mod4/AFE_control/afe_control/phase_compensation_1 ==
  local_time : Inport
  master_time : Inport  Port=2
  Zero-Order Hold : ZeroOrderHold  SampleTime=-1
  Zero-Order Hold1 : ZeroOrderHold  SampleTime=-1
  alignment_eval_afe1 : Subsystem
  y : Outport
  wires:
  Zero-Order Hold1/1 -> alignment_eval_afe1/2(master_time)
  Zero-Order Hold/1 -> alignment_eval_afe1/1(local_time)
  alignment_eval_afe1/1(dp) -> y/1
  master_time/1 -> Zero-Order Hold1/1
  local_time/1 -> Zero-Order Hold/1

== system grid_afe_n/afe_abc_mod4/AFE_control/afe_control/space_vector ==
  uab_out : Inport
  Bus Creator : BusCreator  Inputs=3
  Bus Selector : BusSelector  OutputSignals=da,db,dc
  Bus Selector1 : BusSelector  OutputSignals=ualpha_afe,ubeta_afe,ugamma_afe
  C Caller : CCaller  FunctionName=sv_pwm_cm_process_simulink  PortSpecificationStruct="%)30     .    B H   8    (     @         %    \"     8    !     0         %  0 \"0    $    _    07)G3F%M90  4&]R=$YA;64 4V-O<&4     26YD97@     5'EP90      4VEZ90      27-';&]B86P   X    P    !@    @    $          4    (     0    ,    !         !   P!O=70 #@   #     &    \"     0         !0    @    !     P    $         $  # &]U=  .    .     8    (    !          %    \"     $    &     0         0   ...(+3252 chars)"
  Constant : Constant  Value=glb_time.ts_afe
  Constant1 : Constant
  Data Type Conversion1 : DataTypeConversion  OutDataTypeStr=double  SaturateOnIntegerOverflow=off  RndMeth=Floor
  Data Type Conversion{4,15..16,18} (4 alike) : DataTypeConversion  OutDataTypeStr=single  SaturateOnIntegerOverflow=off  RndMeth=Floor
  Data Type Conversion17 : DataTypeConversion  OutDataTypeStr=uint32  SaturateOnIntegerOverflow=off  RndMeth=Floor
  Data Type Conversion2 : DataTypeConversion  OutDataTypeStr=double  SaturateOnIntegerOverflow=off  RndMeth=Floor
  Data Type Conversion3 : DataTypeConversion  OutDataTypeStr=double  SaturateOnIntegerOverflow=off  RndMeth=Floor
  Gain1 : Gain  Gain=sqrt(3)/2
  Gain2 : Gain  Gain=sqrt(3)/2
  Gain3 : Gain  Gain=u_cm_comp_mod4
  duvw : Outport
  wires:
  Data Type Conversion4/1 -> C Caller/3
  Gain3/1 -> Data Type Conversion4/1
  Bus Selector1/3 -> Gain3/1  "<ugamma_afe>"
  Data Type Conversion17/1 -> C Caller/5
  Data Type Conversion16/1 -> C Caller/4
  Constant1/1 -> Data Type Conversion17/1
  uab_out/1 -> Bus Selector1/1
  Constant/1 -> Data Type Conversion16/1
  Data Type Conversion3/1 -> Bus Creator/3  "dw(k)"
  Gain1/1 -> Data Type Conversion18/1
  Bus Selector/1 -> Data Type Conversion1/1  "<da>"
  Gain2/1 -> Data Type Conversion15/1
  Data Type Conversion2/1 -> Bus Creator/2  "dv(k)"
  Bus Selector1/1 -> Gain1/1  "<ualpha_afe>"
  Bus Selector/3 -> Data Type Conversion3/1  "<dc>"
  Bus Selector1/2 -> Gain2/1  "<ubeta_afe>"
  Data Type Conversion1/1 -> Bus Creator/1  "du(k)"
  Bus Creator/1 -> duvw/1
  C Caller/1 -> Bus Selector/1
  Data Type Conversion18/1 -> C Caller/1
  Bus Selector/2 -> Data Type Conversion2/1  "<db>"
  Data Type Conversion15/1 -> C Caller/2

== system grid_afe_n/afe_abc_mod4/AFE_control/afe_control/udc_acquisition ==
  udc_pu : Inport
  Quantizer : Quantizer  QuantizationInterval=adc_quantization
  Unit Delay : UnitDelay  SampleTime=-1
  Zero-Order Hold : ZeroOrderHold  SampleTime=-1
  udcd_pu : Outport
  wires:
  Zero-Order Hold/1 -> Quantizer/1
  Unit Delay/1 -> udcd_pu/1
  udc_pu/1 -> Zero-Order Hold/1
  Quantizer/1 -> Unit Delay/1

== system grid_afe_n/afe_abc_mod4/AFE_control/afe_control/udc_ctrl ==
  udc_pu : Inport
  udc_pu_ref : Inport  Port=2
  1/Ti : Gain  Gain=afe_ctrl.kp_udc_ctrl  SaturateOnIntegerOverflow=on  OutDataTypeStr=Inherit: Same as input  ParamDataTypeStr=Inherit: Same as input
  Constant : Constant  Value=0
  Gain : Gain  Gain=-1
  Saturation : Saturate  UpperLimit=afe_ctrl.ixi_pos_ref_lim  LowerLimit=-afe_ctrl.ixi_pos_ref_lim
  Sum1 : Sum  Inputs=+++  SaturateOnIntegerOverflow=on
  Sum2 : Sum  Inputs=-+  SaturateOnIntegerOverflow=on
  Sum3 : Sum  Inputs=-+  SaturateOnIntegerOverflow=on
  Switch : Switch  Criteria=u2 > Threshold  SaturateOnIntegerOverflow=off  InputSameDT=off
  To Workspace1 : ToWorkspace  VariableName=udc_pu_sim_mod1  SampleTime=-1
      settings: MaxDataPoints=glb_time.Ns_afe
  To Workspace3 : ToWorkspace  VariableName=udc_pu_ref_sim_mod1  SampleTime=-1
      settings: MaxDataPoints=glb_time.Ns_afe
  Unit Delay4 : UnitDelay  SampleTime=-1
  kp : Gain  Gain=afe_ctrl.ki_udc_ctrl*glb_time.ts_afe  SaturateOnIntegerOverflow=on  OutDataTypeStr=Inherit: Same as input  ParamDataTypeStr=Inherit: Same as input
  udc_tracking : Scope  NumInputPorts=2
      settings: ActiveDisplayYMinimum=-0.14752197265624997  ActiveDisplayYMaximum=1.32769775390625  DataLoggingVariableName=ScopeData8
  i_xi_ref : Outport
  wires:
  Gain/1 -> i_xi_ref/1
  Constant/1 -> Switch/1
  Switch/1 -> Gain/1, Sum3/2
  Saturation/1 -> Switch/3
  [pwr_lim_enable] -> Switch/2
  Sum1/1 -> Saturation/1
  Sum2/1 -> 1/Ti/1, kp/1
  udc_pu/1 -> Sum2/1, udc_tracking/2, To Workspace1/1  "udc_pu"
  udc_pu_ref/1 -> Sum2/2, udc_tracking/1, To Workspace3/1  "udc_pu_ref"
  Unit Delay4/1 -> Sum1/3
  Sum3/1 -> Unit Delay4/1
  kp/1 -> Sum1/2
  1/Ti/1 -> Sum3/1, Sum1/1

== system grid_afe_n/afe_abc_mod4/AFE_control/afe_control/ug afe quantizzation and one step delay ==
  ug_abc_pu : Inport
  Demux : Demux  Outputs=3
  Mux : Mux  Inputs=3
  ug afe quantizzation and one step delay : Subsystem
  ugd_abc_pu : Outport
  wires:
  Mux/1 -> ugd_abc_pu/1
  ug afe quantizzation and one step delay/3(ugd_w_pu) -> Mux/3
  ug_abc_pu/1 -> Demux/1
  Demux/1 -> ug afe quantizzation and one step delay/1(ug_u_pu)
  ug afe quantizzation and one step delay/1(ugd_u_pu) -> Mux/1
  Demux/3 -> ug afe quantizzation and one step delay/3(ug_w_pu)
  Demux/2 -> ug afe quantizzation and one step delay/2(ug_v_pu)
  ug afe quantizzation and one step delay/2(ugd_v_pu) -> Mux/2

== system grid_afe_n/afe_abc_mod4/afe/sv_pwm/modulator1 ==
  u : Inport
  v : Inport  Port=2
  w : Inport  Port=3
  phase : Inport  Port=4
  Bus Creator : BusCreator  Inputs=3
  Three phase two level PWM generator with global TRGO : three_phase_pwm_modulator/Three phase two level PWM generator with global TRGO  f=glb_time.fPWM_AFE  m_up=0.98  m_low=0.02  dead_time=glb_time.dead_time_AFE  pos_cmd_gate=15  neg_cmd_gate=-10  polarity=1  tc=glb_time.tc  double_sampling=1
      link override gate commands/Bus Selector: OutputSignals=du(t)
      link override gate commands/Bus Selector1: OutputSignals=dv(t)
      link override gate commands/Bus Selector2: OutputSignals=dw(t)
  gate_cmds : Outport
  tag scope: TRGO_afe_module_4=global
  wires:
  Three phase two level PWM generator with global TRGO/2 -> gate_cmds/1
  phase/1 -> Three phase two level PWM generator with global TRGO/2
  w/1 -> Bus Creator/3
  v/1 -> Bus Creator/2
  u/1 -> Bus Creator/1
  Three phase two level PWM generator with global TRGO/1 -> [TRGO_afe_module_4]
  Bus Creator/1 -> Three phase two level PWM generator with global TRGO/3
  [time_afe_module_4] -> Three phase two level PWM generator with global TRGO/1

== system grid_afe_n/afe_abc_mod1/AFE_control/afe_control/FRT-VDE4110/FRT-Detection ==
  red_dyn_enabled : Inport
  LVRT_detector : MATLAB Function  TreatAsAtomicUnit=on
  Step1 : Step  Time=0.025  InitialValue=1  FinalValue=0
  Step3 : Step  Time=frt_data.settle_time  FinalValue=frt_data.enable_frt_1 + frt_data.enable_frt_2
  frt_detection_inputs mod1 : Scope  NumInputPorts=6
      settings: ActiveDisplayYMinimum=-1.0098197758197784  ActiveDisplayYMaximum=1.25924351811409  DataLoggingVariableName=ScopeData2
  voltage_rate_measure_neg : Subsystem
  voltage_rate_measure_pos : Subsystem
  frt_exceeded : Outport
  frt_state : Outport  Port=2
  red_dyn_active : Outport  Port=3
  frt_active : Outport  Port=4
  pwr_lim_enable : Outport  Port=5
  wires:
  [v_grid_neg_xi_avg] -> frt_detection_inputs mod1/2, LVRT_detector/2(vxi_n), voltage_rate_measure_neg/1(v_grid_neg_xi_avg)  "v_grid_neg_xi_avg"
  [v_grid_pos_xi_avg] -> voltage_rate_measure_pos/1(v_grid_pos_xi_avg), LVRT_detector/1(vxi_p), frt_detection_inputs mod1/1  "v_grid_pos_xi_avg"
  [v_grid_neg_eta_avg] -> frt_detection_inputs mod1/3, LVRT_detector/3(veta_n)  "v_grid_neg_eta_avg"
  Step3/1 -> frt_detection_inputs mod1/6, LVRT_detector/6(enable)  "enable"
  LVRT_detector/1(pwr_lim_enable) -> pwr_lim_enable/1  "pwr_lim_enable"
  Step1/1 -> LVRT_detector/8(reset)
  red_dyn_enabled/1 -> LVRT_detector/7(red_dyn_enabled)
  LVRT_detector/2(frt_exceeded) -> frt_exceeded/1  "lvrt_exceeded"
  LVRT_detector/5(red_dyn_active) -> red_dyn_active/1
  LVRT_detector/4(frt_state) -> frt_state/1
  LVRT_detector/3(frt_active) -> frt_active/1
  voltage_rate_measure_pos/1(vxi_pos_dot) -> frt_detection_inputs mod1/4, LVRT_detector/4(vxi_p_dot)
  voltage_rate_measure_neg/1(vxi_neg_dot) -> frt_detection_inputs mod1/5, LVRT_detector/5(vxi_n_dot)
